simulink subsystem "SurfEngRef"  (R2024b)
settings: Solver=VariableStepAuto  StartTime=0.0  StopTime=10.0  RelTol=1e-3
undefined symbols (not defined in the file): SimIn, SimPar
libraries: simulink x44, ServosLib x5
(part 2 of 2)

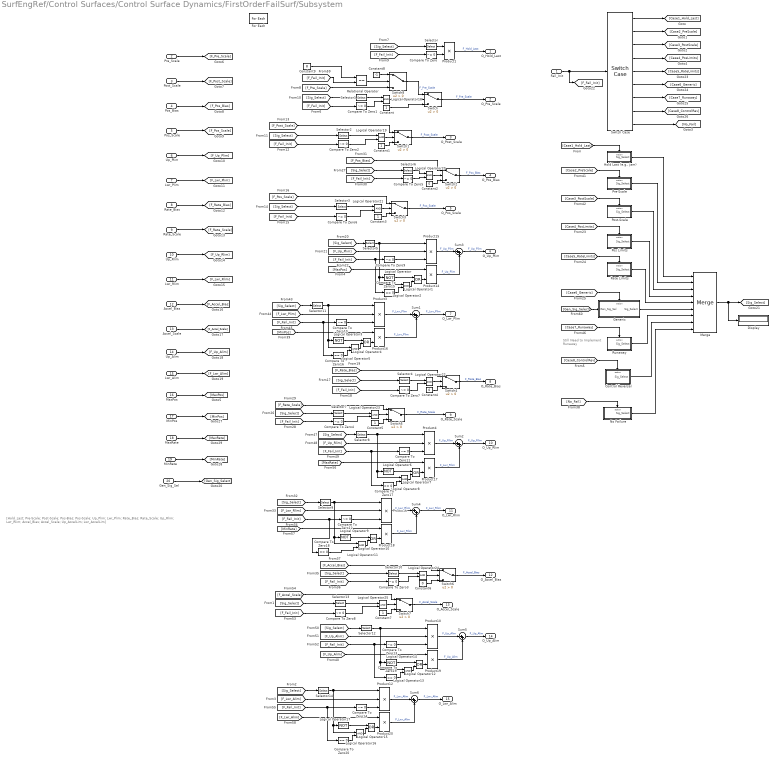
== system SurfEngRef/Control Surfaces/Control Surface Dynamics/FirstOrderFailSurf/Subsystem ==
  note: Still Need to Implement
      | Runaway
  note: [Hold_Last; Pre-Scale; Post-Scale; Pos-Bias; Pos-Scale; Up_Plim; Lwr_Plim; Rate_Bias; Rate_Scale; Up_Rlim; Lwr_Rlim; Accel_Bias; Accel_Scale; Up_AccelLim; Lwr_AccelLim]
  Fail_Init : Inport  Partition=on  PartitionDimension=1  PartitionWidth=1  PartitionOffset=0
  Pre_Scale : Inport  Port=2  Partition=on  PartitionDimension=1  PartitionWidth=1  PartitionOffset=0
  Post_Scale : Inport  Port=3  Partition=on  PartitionDimension=1  PartitionWidth=1  PartitionOffset=0
  Pos_Bias : Inport  Port=4  Partition=on  PartitionDimension=1  PartitionWidth=1  PartitionOffset=0
  Pos_Scale : Inport  Port=5  Partition=on  PartitionDimension=1  PartitionWidth=1  PartitionOffset=0
  Up_Plim : Inport  Port=6  Partition=on  PartitionDimension=1  PartitionWidth=1  PartitionOffset=0
  Lwr_Plim : Inport  Port=7  Partition=on  PartitionDimension=1  PartitionWidth=1  PartitionOffset=0
  Rate_Bias : Inport  Port=8  Partition=on  PartitionDimension=1  PartitionWidth=1  PartitionOffset=0
  Rate_Scale : Inport  Port=9  Partition=on  PartitionDimension=1  PartitionWidth=1  PartitionOffset=0
  Up_Rlim : Inport  Port=10  Partition=on  PartitionDimension=1  PartitionWidth=1  PartitionOffset=0
  Lwr_Rlim : Inport  Port=11  Partition=on  PartitionDimension=1  PartitionWidth=1  PartitionOffset=0
  Accel_Bias : Inport  Port=12  Partition=on  PartitionDimension=1  PartitionWidth=1  PartitionOffset=0
  Accel_Scale : Inport  Port=13  Partition=on  PartitionDimension=1  PartitionWidth=1  PartitionOffset=0
  Up_Alim : Inport  Port=14  Partition=on  PartitionDimension=1  PartitionWidth=1  PartitionOffset=0
  Lwr_Alim : Inport  Port=15  Partition=on  PartitionDimension=1  PartitionWidth=1  PartitionOffset=0
  MaxPos : Inport  Port=16  Partition=on  PartitionDimension=1  PartitionWidth=1  PartitionOffset=0
  MinPos : Inport  Port=17  Partition=on  PartitionDimension=1  PartitionWidth=1  PartitionOffset=0
  MaxRate : Inport  Port=18  Partition=on  PartitionDimension=1  PartitionWidth=1  PartitionOffset=0
  MinRate : Inport  Port=19  Partition=on  PartitionDimension=1  PartitionWidth=1  PartitionOffset=0
  Gen_Sig_Sel : Inport  Port=20
  Compare To Zero{,1..14} (15 alike) : simulink/Logic and Bit Operations/Compare To Zero  relop=~=  OutDataTypeStr=boolean
  Compare To Zero{15..20} (6 alike) : simulink/Logic and Bit Operations/Compare To Zero  relop===  OutDataTypeStr=boolean
  Constant{,1,3,5,7} (5 alike) : Constant
  Constant2 : Constant  Value=0
  Constant4 : Constant  Value=0
  Constant6 : Constant  Value=0
  Constant8 : Constant  Value=-1
  Constant9 : Constant  Value=8
  Control Reversal : Subsystem  TreatAsAtomicUnit=on
  Display : Display
  For Each : ForEach  DisableCoverage=on
  Generic : Subsystem  TreatAsAtomicUnit=on
  "Hold Last (e.g., jam)" : Subsystem  TreatAsAtomicUnit=on
  Logical Operator{,3,6,9,14,17} (6 alike) : Logic  Operator=NOT  AllPortsSameDT=off  OutDataTypeStr=boolean
  Logical Operator{1,4,7,10,12,15} (6 alike) : Logic  Operator=OR  AllPortsSameDT=off  OutDataTypeStr=boolean
  Logical Operator{2,5,8,11,13,16,18..25} (14 alike) : Logic  AllPortsSameDT=off  OutDataTypeStr=boolean
  Merge : Merge  Inputs=9  InitialOutput=7
  No Failure : Subsystem  TreatAsAtomicUnit=on
  Pos Limits : Subsystem  TreatAsAtomicUnit=on
  Post-Scale : Subsystem  TreatAsAtomicUnit=on
  Pre-Scale : Subsystem  TreatAsAtomicUnit=on
  Product{1,14,16..20} (7 alike) : Product
  Product{3..4,6,10,12,15} (6 alike) : Product  Inputs=3
  Rate Limits : Subsystem  TreatAsAtomicUnit=on
  Relational Operator : RelationalOperator  Operator===  OutDataTypeStr=boolean  RndMeth=Simplest  InputSameDT=off
  Runaway : Subsystem  TreatAsAtomicUnit=on
  Selector : Selector  IndexOptions=Index vector (dialog)  Indices=1  OutputSizes=1
  Selector1 : Selector  IndexOptions=Index vector (dialog)  Indices=2  OutputSizes=1
  Selector10 : Selector  IndexOptions=Index vector (dialog)  Indices=12  OutputSizes=1
  Selector11 : Selector  IndexOptions=Index vector (dialog)  Indices=7  OutputSizes=1
  Selector12 : Selector  IndexOptions=Index vector (dialog)  Indices=14  OutputSizes=1
  Selector13 : Selector  IndexOptions=Index vector (dialog)  Indices=13  OutputSizes=1
  Selector14 : Selector  IndexOptions=Index vector (dialog)  Indices=15  OutputSizes=1
  Selector2 : Selector  IndexOptions=Index vector (dialog)  Indices=3  OutputSizes=1
  Selector3 : Selector  IndexOptions=Index vector (dialog)  Indices=5  OutputSizes=1
  Selector4 : Selector  IndexOptions=Index vector (dialog)  Indices=8  OutputSizes=1
  Selector5 : Selector  IndexOptions=Index vector (dialog)  Indices=6  OutputSizes=1
  Selector6 : Selector  IndexOptions=Index vector (dialog)  Indices=4  OutputSizes=1
  Selector7 : Selector  IndexOptions=Index vector (dialog)  Indices=9  OutputSizes=1
  Selector8 : Selector  IndexOptions=Index vector (dialog)  Indices=10  OutputSizes=1
  Selector9 : Selector  IndexOptions=Index vector (dialog)  Indices=11  OutputSizes=1
  Sum{1..6} (6 alike) : Sum  Inputs=|++
  Switch{,1..8} (9 alike) : Switch  Criteria=u2 > Threshold  SaturateOnIntegerOverflow=off  InputSameDT=off
  Switch Case : SwitchCase  CaseConditions={1, 2, 3, 4, 5, 6, 7, 8}
  O_Hold_Last : Outport  ConcatenationDimension=1
  O_Pre_Scale : Outport  Port=2  ConcatenationDimension=1
  O_Post_Scale : Outport  Port=3  ConcatenationDimension=1
  O_Pos_Bias : Outport  Port=4  ConcatenationDimension=1
  O_Pos_Scale : Outport  Port=5  ConcatenationDimension=1
  O_Up_Plim : Outport  Port=6  ConcatenationDimension=1
  O_Lwr_Plim : Outport  Port=7  ConcatenationDimension=1
  O_Rate_Bias : Outport  Port=8  ConcatenationDimension=1
  O_Rate_Scale : Outport  Port=9  ConcatenationDimension=1
  O_Up_Rlim : Outport  Port=10  ConcatenationDimension=1
  O_Lwr_Rlim : Outport  Port=11  ConcatenationDimension=1
  O_Accel_Bias : Outport  Port=12  ConcatenationDimension=1
  O_Accel_Scale : Outport  Port=13  ConcatenationDimension=1
  O_Up_Alim : Outport  Port=14  ConcatenationDimension=1
  O_Lwr_Alim : Outport  Port=15  ConcatenationDimension=1
  wires:
  [Gen_Sig_Select] -> Generic/1(Gen_Sig_Sel)
  Merge/1 -> [Sig_Select], Display/1
  Logical Operator2/1 -> Logical Operator1/2
  Compare To Zero15/1 -> Logical Operator2/2
  Logical Operator1/1 -> Product14/2
  Logical Operator/1 -> Logical Operator1/1
  [MaxPos] -> Product14/1
  Product14/1 -> Sum3/2  "F_Up_Plim"
  Product15/1 -> Sum3/1  "F_Up_Plim"
  MaxRate/1 -> [MaxRate]
  MinRate/1 -> [MinRate]
  MinPos/1 -> [MinPos]
  MaxPos/1 -> [MaxPos]
  [Sig_Select] -> Selector14/1
  [F_Lwr_Alim] -> Product12/2
  [F_Accel_Scale] -> Switch7/1
  [F_Fail_Init] -> Compare To Zero8/1
  Compare To Zero8/1 -> Logical Operator25/2
  Selector13/1 -> Logical Operator25/1
  [Sig_Select] -> Selector13/1
  Selector10/1 -> Logical Operator24/1
  [Sig_Select] -> Selector10/1
  [F_Fail_Init] -> Compare To Zero3/1
  Compare To Zero3/1 -> Logical Operator24/2
  [F_Up_Alim] -> Product10/2
  [Sig_Select] -> Selector12/1
  [F_Accel_Bias] -> Switch6/1
  [F_Lwr_Rlim] -> Product6/2
  [Sig_Select] -> Selector9/1
  [F_Fail_Init] -> Compare To Zero17/1, Compare To Zero11/1
  [Sig_Select] -> Selector8/1
  Switch5/1 -> O_Rate_Scale/1  "F_Rate_Scale"
  [F_Rate_Scale] -> Switch5/1
  Compare To Zero4/1 -> Logical Operator23/2
  [Sig_Select] -> Selector7/1
  Selector7/1 -> Logical Operator23/1
  [F_Fail_Init] -> Compare To Zero4/1
  Switch4/1 -> O_Rate_Bias/1  "F_Rate_Bias"
  [F_Rate_Bias] -> Switch4/1
  Selector4/1 -> Logical Operator22/1
  [Sig_Select] -> Selector4/1
  Compare To Zero7/1 -> Logical Operator22/2
  [F_Fail_Init] -> Compare To Zero7/1
  [F_Fail_Init] -> Compare To Zero6/1
  Compare To Zero6/1 -> Logical Operator21/2
  [Sig_Select] -> Selector3/1
  Selector3/1 -> Logical Operator21/1
  [F_Pos_Scale] -> Switch3/1
  Switch2/1 -> O_Pos_Bias/1  "F_Pos_Bias"
  [Sig_Select] -> Selector6/1
  Selector6/1 -> Logical Operator20/1
  Compare To Zero5/1 -> Logical Operator20/2
  [F_Fail_Init] -> Compare To Zero5/1
  [F_Pos_Bias] -> Switch2/1
  Compare To Zero2/1 -> Logical Operator19/2
  Compare To Zero1/1 -> Logical Operator18/2
  Generic/1(Sig_Select) -> Merge/6
  Runaway/1(Sig_Select) -> Merge/7
  [Case7_Runaway] -> Runaway/Action
  [Case6_Generic] -> Generic/Action
  No Failure/1(Sig_Select) -> Merge/9
  [No_Fail] -> No Failure/Action
  Switch6/1 -> O_Accel_Bias/1  "F_Accel_Bias"
  "Hold Last (e.g., jam)"/1(Sig_Select) -> Merge/1
  Product6/1 -> Sum4/1  "F_Lwr_Rlim"
  Product4/1 -> Sum2/1  "F_Up_Rlim"
  Product3/1 -> Sum1/1  "F_Lwr_Plim"
  Selector5/1 -> Product15/1, Logical Operator/1, Logical Operator2/1
  [Sig_Select] -> Selector5/1
  [F_Up_Plim] -> Product15/2
  Sum3/1 -> O_Up_Plim/1  "F_Up_Plim"
  Switch3/1 -> O_Pos_Scale/1  "F_Pos_Scale"
  Switch1/1 -> O_Post_Scale/1  "F_Post_Scale"
  Selector1/1 -> Logical Operator18/1
  [Sig_Select] -> Selector1/1
  [F_Pre_Scale] -> Switch8/3
  Switch/1 -> O_Pre_Scale/1  "F_Pre_Scale"
  [Sig_Select] -> Selector/1
  Product1/1 -> O_Hold_Last/1  "F_Hold_Last"
  Selector/1 -> Product1/1
  Product12/1 -> Sum6/1  "F_Lwr_Alim"
  Switch7/1 -> O_Accel_Scale/1  "F_Accel_Scale"
  Lwr_Alim/1 -> [F_Lwr_Alim]
  Up_Alim/1 -> [F_Up_Alim]
  Accel_Scale/1 -> [F_Accel_Scale]
  Accel_Bias/1 -> [F_Accel_Bias]
  Lwr_Rlim/1 -> [F_Lwr_Rlim]
  Up_Rlim/1 -> [F_Up_Rlim]
  Rate_Scale/1 -> [F_Rate_Scale]
  Rate_Bias/1 -> [F_Rate_Bias]
  Lwr_Plim/1 -> [F_Lwr_Plim]
  Up_Plim/1 -> [F_Up_Plim]
  Pos_Scale/1 -> [F_Pos_Scale]
  Pos_Bias/1 -> [F_Pos_Bias]
  Post_Scale/1 -> [F_Post_Scale]
  Pre_Scale/1 -> [F_Pre_Scale]
  Switch Case/9 -> [No_Fail]
  [Case1_Hold_Last] -> "Hold Last (e.g., jam)"/Action
  Switch Case/1 -> [Case1_Hold_Last]
  Fail_Init/1 -> [F_Fail_Init], Switch Case/1
  Switch Case/2 -> [Case2_PreScale]
  Switch Case/3 -> [Case3_PostScale]
  Switch Case/4 -> [Case4_PosLimits]
  Switch Case/5 -> [Case5_RateLimits]
  Switch Case/6 -> [Case6_Generic]
  Switch Case/7 -> [Case7_Runaway]
  Switch Case/8 -> [Case8_ControlRev]
  [Case8_ControlRev] -> Control Reversal/Action
  Control Reversal/1(Sig_Select) -> Merge/8
  [Case2_PreScale] -> Pre-Scale/Action
  Compare To Zero/1 -> Product1/2
  [F_Fail_Init] -> Compare To Zero/1
  [F_Fail_Init] -> Compare To Zero1/1
  [F_Fail_Init] -> Compare To Zero2/1
  [Sig_Select] -> Selector2/1
  Selector2/1 -> Logical Operator19/1
  [F_Post_Scale] -> Switch1/1
  Post-Scale/1(Sig_Select) -> Merge/3
  [Case3_PostScale] -> Post-Scale/Action
  Pre-Scale/1(Sig_Select) -> Merge/2
  [F_Fail_Init] -> Compare To Zero9/1, Compare To Zero15/1
  [F_Fail_Init] -> Compare To Zero16/1, Compare To Zero10/1
  [Sig_Select] -> Selector11/1
  [Case4_PosLimits] -> Pos Limits/Action
  Pos Limits/1(Sig_Select) -> Merge/4
  [Case5_RateLimits] -> Rate Limits/Action
  Rate Limits/1(Sig_Select) -> Merge/5
  [F_Lwr_Plim] -> Product3/2
  [F_Up_Rlim] -> Product4/2
  Compare To Zero9/1 -> Product15/3
  Compare To Zero11/1 -> Product4/3
  Compare To Zero12/1 -> Product6/3
  Compare To Zero13/1 -> Product10/3
  Compare To Zero14/1 -> Product12/3
  Product10/1 -> Sum5/1  "F_Up_Alim"
  Compare To Zero10/1 -> Product3/3
  Selector11/1 -> Logical Operator3/1, Logical Operator5/1, Product3/1
  Logical Operator5/1 -> Logical Operator4/2
  Compare To Zero16/1 -> Logical Operator5/2
  Logical Operator3/1 -> Logical Operator4/1
  Logical Operator4/1 -> Product16/2
  [MinPos] -> Product16/1
  Product16/1 -> Sum1/2  "F_Lwr_Plim"
  Sum1/1 -> O_Lwr_Plim/1  "F_Lwr_Plim"
  Logical Operator7/1 -> Product17/2
  Logical Operator6/1 -> Logical Operator7/1
  Selector8/1 -> Logical Operator6/1, Logical Operator8/1, Product4/1
  Compare To Zero17/1 -> Logical Operator8/2
  Logical Operator8/1 -> Logical Operator7/2
  Sum2/1 -> O_Up_Rlim/1  "F_Up_Rlim"
  Product17/1 -> Sum2/2  "F_Lwr_Rlim"
  [MaxRate] -> Product17/1
  Compare To Zero18/1 -> Logical Operator11/2
  Product18/1 -> Sum4/2  "F_Lwr_Rlim"
  Logical Operator9/1 -> Logical Operator10/1
  Logical Operator10/1 -> Product18/2
  [F_Fail_Init] -> Compare To Zero18/1, Compare To Zero12/1
  Selector9/1 -> Logical Operator9/1, Logical Operator11/1, Product6/1
  Logical Operator11/1 -> Logical Operator10/2
  Sum4/1 -> O_Lwr_Rlim/1  "F_Lwr_Rlim"
  [MinRate] -> Product18/1
  Logical Operator13/1 -> Logical Operator12/2
  Logical Operator12/1 -> Product19/2
  Logical Operator14/1 -> Logical Operator12/1
  [F_Fail_Init] -> Compare To Zero19/1, Compare To Zero13/1
  Selector12/1 -> Logical Operator14/1, Logical Operator13/1, Product10/1
  Compare To Zero19/1 -> Logical Operator13/2
  Sum5/1 -> O_Up_Alim/1  "F_Up_Alim"
  [F_Up_Alim] -> Product19/1
  Selector14/1 -> Logical Operator17/1, Logical Operator16/1, Product12/1
  Logical Operator17/1 -> Logical Operator15/1
  Logical Operator16/1 -> Logical Operator15/2
  Compare To Zero20/1 -> Logical Operator16/2
  [F_Fail_Init] -> Compare To Zero20/1, Compare To Zero14/1
  Logical Operator15/1 -> Product20/2
  Sum6/1 -> O_Lwr_Alim/1  "F_Lwr_Alim"
  Product20/1 -> Sum6/2  "F_Lwr_Alim"
  [F_Lwr_Alim] -> Product20/1
  Product19/1 -> Sum5/2  "F_Up_Alim"
  Logical Operator18/1 -> Switch/2
  Constant/1 -> Switch/3
  Logical Operator19/1 -> Switch1/2
  Constant1/1 -> Switch1/3
  Constant2/1 -> Switch2/3
  Logical Operator20/1 -> Switch2/2
  Constant3/1 -> Switch3/3
  Logical Operator21/1 -> Switch3/2
  Logical Operator22/1 -> Switch4/2
  Constant4/1 -> Switch4/3
  Logical Operator23/1 -> Switch5/2
  Constant5/1 -> Switch5/3
  Logical Operator24/1 -> Switch6/2
  Constant6/1 -> Switch6/3
  Logical Operator25/1 -> Switch7/2
  Constant7/1 -> Switch7/3
  Switch8/1 -> Switch/1  "F_Pre_Scale"
  Constant8/1 -> Switch8/1
  [F_Fail_Init] -> Relational Operator/2
  Relational Operator/1 -> Switch8/2
  Constant9/1 -> Relational Operator/1
  Gen_Sig_Sel/1 -> [Gen_Sig_Select]

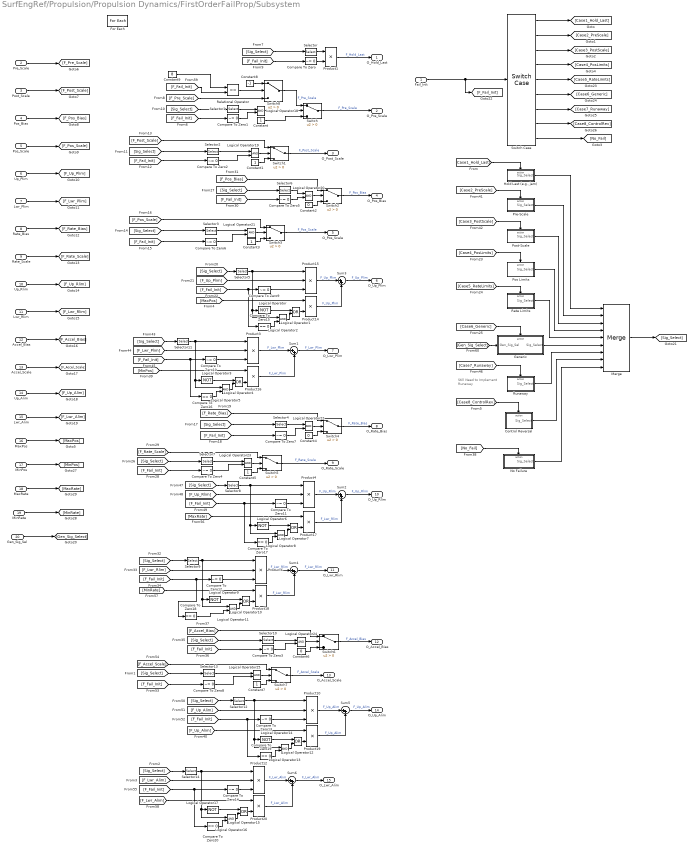
== system SurfEngRef/Propulsion/Propulsion Dynamics/FirstOrderFailProp/Subsystem ==
  note: Still Need to Implement
      | Runaway
  Fail_Init : Inport  Partition=on  PartitionDimension=1  PartitionWidth=1  PartitionOffset=0
  Pre_Scale : Inport  Port=2  Partition=on  PartitionDimension=1  PartitionWidth=1  PartitionOffset=0
  Post_Scale : Inport  Port=3  Partition=on  PartitionDimension=1  PartitionWidth=1  PartitionOffset=0
  Pos_Bias : Inport  Port=4  Partition=on  PartitionDimension=1  PartitionWidth=1  PartitionOffset=0
  Pos_Scale : Inport  Port=5  Partition=on  PartitionDimension=1  PartitionWidth=1  PartitionOffset=0
  Up_Plim : Inport  Port=6  Partition=on  PartitionDimension=1  PartitionWidth=1  PartitionOffset=0
  Lwr_Plim : Inport  Port=7  Partition=on  PartitionDimension=1  PartitionWidth=1  PartitionOffset=0
  Rate_Bias : Inport  Port=8  Partition=on  PartitionDimension=1  PartitionWidth=1  PartitionOffset=0
  Rate_Scale : Inport  Port=9  Partition=on  PartitionDimension=1  PartitionWidth=1  PartitionOffset=0
  Up_Rlim : Inport  Port=10  Partition=on  PartitionDimension=1  PartitionWidth=1  PartitionOffset=0
  Lwr_Rlim : Inport  Port=11  Partition=on  PartitionDimension=1  PartitionWidth=1  PartitionOffset=0
  Accel_Bias : Inport  Port=12  Partition=on  PartitionDimension=1  PartitionWidth=1  PartitionOffset=0
  Accel_Scale : Inport  Port=13  Partition=on  PartitionDimension=1  PartitionWidth=1  PartitionOffset=0
  Up_Alim : Inport  Port=14  Partition=on  PartitionDimension=1  PartitionWidth=1  PartitionOffset=0
  Lwr_Alim : Inport  Port=15  Partition=on  PartitionDimension=1  PartitionWidth=1  PartitionOffset=0
  MaxPos : Inport  Port=16  Partition=on  PartitionDimension=1  PartitionWidth=1  PartitionOffset=0
  MinPos : Inport  Port=17  Partition=on  PartitionDimension=1  PartitionWidth=1  PartitionOffset=0
  MaxRate : Inport  Port=18  Partition=on  PartitionDimension=1  PartitionWidth=1  PartitionOffset=0
  MinRate : Inport  Port=19  Partition=on  PartitionDimension=1  PartitionWidth=1  PartitionOffset=0
  Gen_Sig_Sel : Inport  Port=20
  Compare To Zero{,1..14} (15 alike) : simulink/Logic and Bit Operations/Compare To Zero  relop=~=  OutDataTypeStr=boolean
  Compare To Zero{15..20} (6 alike) : simulink/Logic and Bit Operations/Compare To Zero  relop===  OutDataTypeStr=boolean
  Constant{,1,3,5,7} (5 alike) : Constant
  Constant2 : Constant  Value=0
  Constant4 : Constant  Value=0
  Constant6 : Constant  Value=0
  Constant8 : Constant  Value=-1
  Constant9 : Constant  Value=8
  Control Reversal : Subsystem  TreatAsAtomicUnit=on
  For Each : ForEach  DisableCoverage=on
  Generic : Subsystem  TreatAsAtomicUnit=on
  "Hold Last (e.g., jam)" : Subsystem  TreatAsAtomicUnit=on
  Logical Operator{,3,6,9,14,17} (6 alike) : Logic  Operator=NOT  AllPortsSameDT=off  OutDataTypeStr=boolean
  Logical Operator{1,4,7,10,12,15} (6 alike) : Logic  Operator=OR  AllPortsSameDT=off  OutDataTypeStr=boolean
  Logical Operator{2,5,8,11,13,16,18..25} (14 alike) : Logic  AllPortsSameDT=off  OutDataTypeStr=boolean
  Merge : Merge  Inputs=9
  No Failure : Subsystem  TreatAsAtomicUnit=on
  Pos Limits : Subsystem  TreatAsAtomicUnit=on
  Post-Scale : Subsystem  TreatAsAtomicUnit=on
  Pre-Scale : Subsystem  TreatAsAtomicUnit=on
  Product{1,14,16..20} (7 alike) : Product
  Product{3..4,6,10,12,15} (6 alike) : Product  Inputs=3
  Rate Limits : Subsystem  TreatAsAtomicUnit=on
  Relational Operator : RelationalOperator  Operator===  OutDataTypeStr=boolean  RndMeth=Simplest  InputSameDT=off
  Runaway : Subsystem  TreatAsAtomicUnit=on
  Selector : Selector  IndexOptions=Index vector (dialog)  Indices=1  OutputSizes=1
  Selector1 : Selector  IndexOptions=Index vector (dialog)  Indices=2  OutputSizes=1
  Selector10 : Selector  IndexOptions=Index vector (dialog)  Indices=12  OutputSizes=1
  Selector11 : Selector  IndexOptions=Index vector (dialog)  Indices=7  OutputSizes=1
  Selector12 : Selector  IndexOptions=Index vector (dialog)  Indices=14  OutputSizes=1
  Selector13 : Selector  IndexOptions=Index vector (dialog)  Indices=13  OutputSizes=1
  Selector14 : Selector  IndexOptions=Index vector (dialog)  Indices=15  OutputSizes=1
  Selector2 : Selector  IndexOptions=Index vector (dialog)  Indices=3  OutputSizes=1
  Selector3 : Selector  IndexOptions=Index vector (dialog)  Indices=5  OutputSizes=1
  Selector4 : Selector  IndexOptions=Index vector (dialog)  Indices=8  OutputSizes=1
  Selector5 : Selector  IndexOptions=Index vector (dialog)  Indices=6  OutputSizes=1
  Selector6 : Selector  IndexOptions=Index vector (dialog)  Indices=4  OutputSizes=1
  Selector7 : Selector  IndexOptions=Index vector (dialog)  Indices=9  OutputSizes=1
  Selector8 : Selector  IndexOptions=Index vector (dialog)  Indices=10  OutputSizes=1
  Selector9 : Selector  IndexOptions=Index vector (dialog)  Indices=11  OutputSizes=1
  Sum{1..6} (6 alike) : Sum  Inputs=|++
  Switch{,1..8} (9 alike) : Switch  Criteria=u2 > Threshold  SaturateOnIntegerOverflow=off  InputSameDT=off
  Switch Case : SwitchCase  CaseConditions={1, 2, 3, 4, 5, 6, 7, 8}
  O_Hold_Last : Outport  ConcatenationDimension=1
  O_Pre_Scale : Outport  Port=2  ConcatenationDimension=1
  O_Post_Scale : Outport  Port=3  ConcatenationDimension=1
  O_Pos_Bias : Outport  Port=4  ConcatenationDimension=1
  O_Pos_Scale : Outport  Port=5  ConcatenationDimension=1
  O_Up_Plim : Outport  Port=6  ConcatenationDimension=1
  O_Lwr_Plim : Outport  Port=7  ConcatenationDimension=1
  O_Rate_Bias : Outport  Port=8  ConcatenationDimension=1
  O_Rate_Scale : Outport  Port=9  ConcatenationDimension=1
  O_Up_Rlim : Outport  Port=10  ConcatenationDimension=1
  O_Lwr_Rlim : Outport  Port=11  ConcatenationDimension=1
  O_Accel_Bias : Outport  Port=12  ConcatenationDimension=1
  O_Accel_Scale : Outport  Port=13  ConcatenationDimension=1
  O_Up_Alim : Outport  Port=14  ConcatenationDimension=1
  O_Lwr_Alim : Outport  Port=15  ConcatenationDimension=1
  wires:
  Gen_Sig_Sel/1 -> [Gen_Sig_Select]
  [Gen_Sig_Select] -> Generic/1(Gen_Sig_Sel)
  Merge/1 -> [Sig_Select]
  Logical Operator2/1 -> Logical Operator1/2
  Compare To Zero15/1 -> Logical Operator2/2
  Logical Operator1/1 -> Product14/2
  Logical Operator/1 -> Logical Operator1/1
  [MaxPos] -> Product14/1
  Product14/1 -> Sum3/2  "F_Up_Plim"
  Product15/1 -> Sum3/1  "F_Up_Plim"
  MaxRate/1 -> [MaxRate]
  MinRate/1 -> [MinRate]
  MinPos/1 -> [MinPos]
  MaxPos/1 -> [MaxPos]
  [Sig_Select] -> Selector14/1
  [F_Lwr_Alim] -> Product12/2
  [F_Accel_Scale] -> Switch7/1
  [F_Fail_Init] -> Compare To Zero8/1
  Compare To Zero8/1 -> Logical Operator25/2
  Selector13/1 -> Logical Operator25/1
  [Sig_Select] -> Selector13/1
  Selector10/1 -> Logical Operator24/1
  [Sig_Select] -> Selector10/1
  [F_Fail_Init] -> Compare To Zero3/1
  Compare To Zero3/1 -> Logical Operator24/2
  [F_Up_Alim] -> Product10/2
  [Sig_Select] -> Selector12/1
  [F_Accel_Bias] -> Switch6/1
  [F_Lwr_Rlim] -> Product6/2
  [Sig_Select] -> Selector9/1
  [F_Fail_Init] -> Compare To Zero17/1, Compare To Zero11/1
  [Sig_Select] -> Selector8/1
  Switch5/1 -> O_Rate_Scale/1  "F_Rate_Scale"
  [F_Rate_Scale] -> Switch5/1
  Compare To Zero4/1 -> Logical Operator23/2
  [Sig_Select] -> Selector7/1
  Selector7/1 -> Logical Operator23/1
  [F_Fail_Init] -> Compare To Zero4/1
  Switch4/1 -> O_Rate_Bias/1  "F_Rate_Bias"
  [F_Rate_Bias] -> Switch4/1
  Selector4/1 -> Logical Operator22/1
  [Sig_Select] -> Selector4/1
  Compare To Zero7/1 -> Logical Operator22/2
  [F_Fail_Init] -> Compare To Zero7/1
  [F_Fail_Init] -> Compare To Zero6/1
  Compare To Zero6/1 -> Logical Operator21/2
  [Sig_Select] -> Selector3/1
  Selector3/1 -> Logical Operator21/1
  [F_Pos_Scale] -> Switch3/1
  Switch2/1 -> O_Pos_Bias/1  "F_Pos_Bias"
  [Sig_Select] -> Selector6/1
  Selector6/1 -> Logical Operator20/1
  Compare To Zero5/1 -> Logical Operator20/2
  [F_Fail_Init] -> Compare To Zero5/1
  [F_Pos_Bias] -> Switch2/1
  Compare To Zero2/1 -> Logical Operator19/2
  Compare To Zero1/1 -> Logical Operator18/2
  Generic/1(Sig_Select) -> Merge/6
  Runaway/1(Sig_Select) -> Merge/7
  [Case7_Runaway] -> Runaway/Action
  [Case6_Generic] -> Generic/Action
  No Failure/1(Sig_Select) -> Merge/9
  [No_Fail] -> No Failure/Action
  Switch6/1 -> O_Accel_Bias/1  "F_Accel_Bias"
  "Hold Last (e.g., jam)"/1(Sig_Select) -> Merge/1
  Product6/1 -> Sum4/1  "F_Lwr_Rlim"
  Product4/1 -> Sum2/1  "F_Up_Rlim"
  Product3/1 -> Sum1/1  "F_Lwr_Plim"
  Selector5/1 -> Product15/1, Logical Operator/1, Logical Operator2/1
  [Sig_Select] -> Selector5/1
  [F_Up_Plim] -> Product15/2
  Sum3/1 -> O_Up_Plim/1  "F_Up_Plim"
  Switch3/1 -> O_Pos_Scale/1  "F_Pos_Scale"
  Switch1/1 -> O_Post_Scale/1  "F_Post_Scale"
  Selector1/1 -> Logical Operator18/1
  [Sig_Select] -> Selector1/1
  [F_Pre_Scale] -> Switch8/3
  Switch/1 -> O_Pre_Scale/1  "F_Pre_Scale"
  [Sig_Select] -> Selector/1
  Product1/1 -> O_Hold_Last/1  "F_Hold_Last"
  Selector/1 -> Product1/1
  Product12/1 -> Sum6/1  "F_Lwr_Alim"
  Switch7/1 -> O_Accel_Scale/1  "F_Accel_Scale"
  Lwr_Alim/1 -> [F_Lwr_Alim]
  Up_Alim/1 -> [F_Up_Alim]
  Accel_Scale/1 -> [F_Accel_Scale]
  Accel_Bias/1 -> [F_Accel_Bias]
  Lwr_Rlim/1 -> [F_Lwr_Rlim]
  Up_Rlim/1 -> [F_Up_Rlim]
  Rate_Scale/1 -> [F_Rate_Scale]
  Rate_Bias/1 -> [F_Rate_Bias]
  Lwr_Plim/1 -> [F_Lwr_Plim]
  Up_Plim/1 -> [F_Up_Plim]
  Pos_Scale/1 -> [F_Pos_Scale]
  Pos_Bias/1 -> [F_Pos_Bias]
  Post_Scale/1 -> [F_Post_Scale]
  Pre_Scale/1 -> [F_Pre_Scale]
  Switch Case/9 -> [No_Fail]
  [Case1_Hold_Last] -> "Hold Last (e.g., jam)"/Action
  Switch Case/1 -> [Case1_Hold_Last]
  Fail_Init/1 -> [F_Fail_Init], Switch Case/1
  Switch Case/2 -> [Case2_PreScale]
  Switch Case/3 -> [Case3_PostScale]
  Switch Case/4 -> [Case4_PosLimits]
  Switch Case/5 -> [Case5_RateLimits]
  Switch Case/6 -> [Case6_Generic]
  Switch Case/7 -> [Case7_Runaway]
  Switch Case/8 -> [Case8_ControlRev]
  [Case8_ControlRev] -> Control Reversal/Action
  Control Reversal/1(Sig_Select) -> Merge/8
  [Case2_PreScale] -> Pre-Scale/Action
  Compare To Zero/1 -> Product1/2
  [F_Fail_Init] -> Compare To Zero/1
  [F_Fail_Init] -> Compare To Zero1/1
  [F_Fail_Init] -> Compare To Zero2/1
  [Sig_Select] -> Selector2/1
  Selector2/1 -> Logical Operator19/1
  [F_Post_Scale] -> Switch1/1
  Post-Scale/1(Sig_Select) -> Merge/3
  [Case3_PostScale] -> Post-Scale/Action
  Pre-Scale/1(Sig_Select) -> Merge/2
  [F_Fail_Init] -> Compare To Zero9/1, Compare To Zero15/1
  [F_Fail_Init] -> Compare To Zero16/1, Compare To Zero10/1
  [Sig_Select] -> Selector11/1
  [Case4_PosLimits] -> Pos Limits/Action
  Pos Limits/1(Sig_Select) -> Merge/4
  [Case5_RateLimits] -> Rate Limits/Action
  Rate Limits/1(Sig_Select) -> Merge/5
  [F_Lwr_Plim] -> Product3/2
  [F_Up_Rlim] -> Product4/2
  Compare To Zero9/1 -> Product15/3
  Compare To Zero11/1 -> Product4/3
  Compare To Zero12/1 -> Product6/3
  Compare To Zero13/1 -> Product10/3
  Compare To Zero14/1 -> Product12/3
  Product10/1 -> Sum5/1  "F_Up_Alim"
  Compare To Zero10/1 -> Product3/3
  Selector11/1 -> Logical Operator3/1, Logical Operator5/1, Product3/1
  Logical Operator5/1 -> Logical Operator4/2
  Compare To Zero16/1 -> Logical Operator5/2
  Logical Operator3/1 -> Logical Operator4/1
  Logical Operator4/1 -> Product16/2
  [MinPos] -> Product16/1
  Product16/1 -> Sum1/2  "F_Lwr_Plim"
  Sum1/1 -> O_Lwr_Plim/1  "F_Lwr_Plim"
  Logical Operator7/1 -> Product17/2
  Logical Operator6/1 -> Logical Operator7/1
  Selector8/1 -> Logical Operator6/1, Logical Operator8/1, Product4/1
  Compare To Zero17/1 -> Logical Operator8/2
  Logical Operator8/1 -> Logical Operator7/2
  Sum2/1 -> O_Up_Rlim/1  "F_Up_Rlim"
  Product17/1 -> Sum2/2  "F_Lwr_Rlim"
  [MaxRate] -> Product17/1
  Compare To Zero18/1 -> Logical Operator11/2
  Product18/1 -> Sum4/2  "F_Lwr_Rlim"
  Logical Operator9/1 -> Logical Operator10/1
  Logical Operator10/1 -> Product18/2
  [F_Fail_Init] -> Compare To Zero18/1, Compare To Zero12/1
  Selector9/1 -> Logical Operator9/1, Logical Operator11/1, Product6/1
  Logical Operator11/1 -> Logical Operator10/2
  Sum4/1 -> O_Lwr_Rlim/1  "F_Lwr_Rlim"
  [MinRate] -> Product18/1
  Logical Operator13/1 -> Logical Operator12/2
  Logical Operator12/1 -> Product19/2
  Logical Operator14/1 -> Logical Operator12/1
  [F_Fail_Init] -> Compare To Zero19/1, Compare To Zero13/1
  Selector12/1 -> Logical Operator14/1, Logical Operator13/1, Product10/1
  Compare To Zero19/1 -> Logical Operator13/2
  Sum5/1 -> O_Up_Alim/1  "F_Up_Alim"
  [F_Up_Alim] -> Product19/1
  Selector14/1 -> Logical Operator17/1, Logical Operator16/1, Product12/1
  Logical Operator17/1 -> Logical Operator15/1
  Logical Operator16/1 -> Logical Operator15/2
  Compare To Zero20/1 -> Logical Operator16/2
  [F_Fail_Init] -> Compare To Zero20/1, Compare To Zero14/1
  Logical Operator15/1 -> Product20/2
  Sum6/1 -> O_Lwr_Alim/1  "F_Lwr_Alim"
  Product20/1 -> Sum6/2  "F_Lwr_Alim"
  [F_Lwr_Alim] -> Product20/1
  Product19/1 -> Sum5/2  "F_Up_Alim"
  Logical Operator18/1 -> Switch/2
  Constant/1 -> Switch/3
  Logical Operator19/1 -> Switch1/2
  Constant1/1 -> Switch1/3
  Constant2/1 -> Switch2/3
  Logical Operator20/1 -> Switch2/2
  Constant3/1 -> Switch3/3
  Logical Operator21/1 -> Switch3/2
  Logical Operator22/1 -> Switch4/2
  Constant4/1 -> Switch4/3
  Logical Operator23/1 -> Switch5/2
  Constant5/1 -> Switch5/3
  Logical Operator24/1 -> Switch6/2
  Constant6/1 -> Switch6/3
  Logical Operator25/1 -> Switch7/2
  Constant7/1 -> Switch7/3
  Switch8/1 -> Switch/1  "F_Pre_Scale"
  Constant8/1 -> Switch8/1
  [F_Fail_Init] -> Relational Operator/2
  Relational Operator/1 -> Switch8/2
  Constant9/1 -> Relational Operator/1

== system SurfEngRef/Control Surfaces/Control Surface Dynamics/FirstOrderFailSurf/First Order Dynamic Rate and Position Limited Servo/For Each Subsystem ==
  Cont_Switch : Inport  Partition=on  PartitionDimension=1  PartitionWidth=1  PartitionOffset=0
  pos_in : Inport  Port=2  Partition=on  PartitionDimension=1  PartitionWidth=1  PartitionOffset=0
  For Each : ForEach  DisableCoverage=on
  Memory : Memory
  Switch : Switch  Criteria=u2 ~= 0  SaturateOnIntegerOverflow=off  InputSameDT=off
  pos : Outport  ConcatenationDimension=1
  wires:
  pos_in/1 -> Switch/3
  Cont_Switch/1 -> Switch/2
  Switch/1 -> pos/1, Memory/1
  Memory/1 -> Switch/1

== system SurfEngRef/Control Surfaces/Control Surface Dynamics/FirstOrderFailSurf/Subsystem/Control Reversal ==
  Action Port : ActionPort
  Constant : Constant  Value=[0; 1; zeros(13,1)]
  Sig_Select : Outport
  wires:
  Constant/1 -> Sig_Select/1

== system SurfEngRef/Control Surfaces/Control Surface Dynamics/FirstOrderFailSurf/Subsystem/Generic ==
  Gen_Sig_Sel : Inport
  Action Port : ActionPort
  Sig_Select : Outport
  wires:
  Gen_Sig_Sel/1 -> Sig_Select/1

== system SurfEngRef/Control Surfaces/Control Surface Dynamics/FirstOrderFailSurf/Subsystem/Hold Last (e.g., jam) ==
  note: CASE: Hold Last
      | - Execute hold last on specific effector: e.g., effector jam
      |
      | Outputs:
      | - Sig_Select: column vector (11 elements) of 1s or 0s to specify which output components to overwrite
  Action Port : ActionPort
  Constant : Constant  Value=[1; zeros(14,1)]
  Sig_Select : Outport
  wires:
  Constant/1 -> Sig_Select/1

== system SurfEngRef/Control Surfaces/Control Surface Dynamics/FirstOrderFailSurf/Subsystem/No Failure ==
  note: CASE: Default (No failure)
      |
      | Outputs:
      | - Sig_Select: column vector (11 elements) of all 0s to specify that no outputs should be overwritten
  Action Port : ActionPort
  Constant : Constant  Value=[zeros(15,1)]
  Sig_Select : Outport
  wires:
  Constant/1 -> Sig_Select/1

== system SurfEngRef/Control Surfaces/Control Surface Dynamics/FirstOrderFailSurf/Subsystem/Pos Limits ==
  Action Port : ActionPort
  Constant : Constant  Value=[zeros(3,1); 1; 1; 1; 1; zeros(8,1)]
  Sig_Select : Outport
  wires:
  Constant/1 -> Sig_Select/1

== system SurfEngRef/Control Surfaces/Control Surface Dynamics/FirstOrderFailSurf/Subsystem/Post-Scale ==
  Action Port : ActionPort
  Constant : Constant  Value=[0; 0; 1; zeros(12,1)]
  Sig_Select : Outport
  wires:
  Constant/1 -> Sig_Select/1

== system SurfEngRef/Control Surfaces/Control Surface Dynamics/FirstOrderFailSurf/Subsystem/Pre-Scale ==
  Action Port : ActionPort
  Constant : Constant  Value=[0; 1; zeros(13,1)]
  Sig_Select : Outport
  wires:
  Constant/1 -> Sig_Select/1

== system SurfEngRef/Control Surfaces/Control Surface Dynamics/FirstOrderFailSurf/Subsystem/Rate Limits ==
  Action Port : ActionPort
  Constant : Constant  Value=[zeros(7,1); 1; 1; 1; 1; zeros(4,1)]
  Sig_Select : Outport
  wires:
  Constant/1 -> Sig_Select/1

== system SurfEngRef/Control Surfaces/Control Surface Dynamics/FirstOrderFailSurf/Subsystem/Runaway ==
  note: Runaway currently not implemented
  Action Port : ActionPort
  Constant : Constant  Value=[zeros(15,1)]
  Sig_Select : Outport
  wires:
  Constant/1 -> Sig_Select/1

== system SurfEngRef/Propulsion/Propulsion Dynamics/FirstOrderFailProp/Subsystem/Control Reversal ==
  Action Port : ActionPort
  Constant : Constant  Value=[0; 1; zeros(13,1)]
  Sig_Select : Outport
  wires:
  Constant/1 -> Sig_Select/1

== system SurfEngRef/Propulsion/Propulsion Dynamics/FirstOrderFailProp/Subsystem/Generic ==
  Gen_Sig_Sel : Inport
  Action Port : ActionPort
  Sig_Select : Outport
  wires:
  Gen_Sig_Sel/1 -> Sig_Select/1

== system SurfEngRef/Propulsion/Propulsion Dynamics/FirstOrderFailProp/Subsystem/Hold Last (e.g., jam) ==
  note: CASE: Hold Last
      | - Execute hold last on specific effector: e.g., effector jam
      |
      | Outputs:
      | - Sig_Select: column vector (11 elements) of 1s or 0s to specify which output components to overwrite
  Action Port : ActionPort
  Constant : Constant  Value=[1; zeros(14,1)]
  Sig_Select : Outport
  wires:
  Constant/1 -> Sig_Select/1

== system SurfEngRef/Propulsion/Propulsion Dynamics/FirstOrderFailProp/Subsystem/No Failure ==
  note: CASE: Default (No failure)
      |
      | Outputs:
      | - Sig_Select: column vector (11 elements) of all 0s to specify that no outputs should be overwritten
  Action Port : ActionPort
  Constant : Constant  Value=[zeros(15,1)]
  Sig_Select : Outport
  wires:
  Constant/1 -> Sig_Select/1

== system SurfEngRef/Propulsion/Propulsion Dynamics/FirstOrderFailProp/Subsystem/Pos Limits ==
  Action Port : ActionPort
  Constant : Constant  Value=[zeros(5,1); 1; 1; zeros(8,1)]
  Sig_Select : Outport
  wires:
  Constant/1 -> Sig_Select/1

== system SurfEngRef/Propulsion/Propulsion Dynamics/FirstOrderFailProp/Subsystem/Post-Scale ==
  Action Port : ActionPort
  Constant : Constant  Value=[0; 0; 1; zeros(12,1)]
  Sig_Select : Outport
  wires:
  Constant/1 -> Sig_Select/1

== system SurfEngRef/Propulsion/Propulsion Dynamics/FirstOrderFailProp/Subsystem/Pre-Scale ==
  Action Port : ActionPort
  Constant : Constant  Value=[0; 1; zeros(13,1)]
  Sig_Select : Outport
  wires:
  Constant/1 -> Sig_Select/1

== system SurfEngRef/Propulsion/Propulsion Dynamics/FirstOrderFailProp/Subsystem/Rate Limits ==
  Action Port : ActionPort
  Constant : Constant  Value=[zeros(7,1); 1; 1; zeros(6,1)]
  Sig_Select : Outport
  wires:
  Constant/1 -> Sig_Select/1

== system SurfEngRef/Propulsion/Propulsion Dynamics/FirstOrderFailProp/Subsystem/Runaway ==
  note: Runaway currently not implemented
  Action Port : ActionPort
  Constant : Constant  Value=[zeros(15,1)]
  Sig_Select : Outport
  wires:
  Constant/1 -> Sig_Select/1
